simulink model "XROBO01_reference"  (R2025a)
settings: Solver=ode15s  StartTime=0  StopTime=2.95184041250516  MaxStep=0.002  RelTol=1e-3  AbsTol=1e-4  EnableMultiTasking=on
InitFcn:
  | d2r = pi/180; r2d = 180/pi;
  | assert(exist('initial_forward_speed_mps','var')==1,'XROBO01_PUBLIC_INPUT_MISSING:initial_forward_speed_mps');
  | assert(exist('supported_mass_kg','var')==1,'XROBO01_PUBLIC_INPUT_MISSING:supported_mass_kg');
  | assert(exist('ground_stiffness_npm','var')==1,'XROBO01_PUBLIC_INPUT_MISSING:ground_stiffness_npm');
  | assert(exist('ground_damping_nspm','var')==1,'XROBO01_PUBLIC_INPUT_MISSING:ground_damping_nspm');
  | assert(exist('propulsive_torque_nm','var')==1,'XROBO01_PUBLIC_INPUT_MISSING:propulsive_torque_nm');
  | assert(exist('knee_stiffness_nmprad','var')==1,'XROBO01_PUBLIC_INPUT_MISSING:knee_stiffness_nmprad');
  | u0 = initial_forward_speed_mps; M = supported_mass_kg;
  | ground = struct('stiffness',ground_stiffness_npm,'damping',ground_damping_nspm);
  | Trq_propulsive = propulsive_torque_nm; k2 = knee_stiffness_nmprad;
model workspace (MAT data in the model file):
  DataValues = [0 -8.46607862487e-28 -3.0230079043e-07 -3.0230079043e-07 -0.00122724595841 -0.00736196406339 -0.038035529735 -0.172846716535 -0.307649006025 -0.442435463868 -0.577199164336 -0.711933194065 ... (996 elements, 996x1)]
  F90_INTERNAL_TASK_VERSION = "F90-XROBO-01/INTERNAL_TESTABLE_V0"
  J = 0.317042404181
  L = 1
  L_back = 1.5
  L_stance = 0.85
  N = 80
  T_cg = 0.491973402084
  T_stance = 0.243620261167
  TimeValues = [0 6.27984023631e-30 2.24236125286e-09 2.24236125286e-09 9.10328015658e-06 5.46084691332e-05 0.000282134414016 0.00128213441402 0.00228213441402 0.00328213441402 0.00428213441402 0.00528213441402 ... (996 elements, 996x1)]
  bw = 200
  g = 9.81
  joint_damping = 0.1
  k = 5315
  knee_torque.time = [0 3.68781730895e-05 7.3756346179e-05 0.000110634519268 0.000347975944129 0.00058531736899 0.000822658793851 0.00106000021871 0.00146561022046 0.00187122022221 0.00227683022396 0.00268244022572 ... (1021 elements, 1021x1)]
  knee_torque.signals.values = [0.714762207266 1.14171505645 1.56256115584 1.97723731234 4.51139321024 6.81208984715 8.89224399956 10.7664604725 13.5316206084 15.8030887862 17.6429346124 19.1050336017 ... (1021 elements, 1021x1)]
  knee_torque.signals.dimensions = 1
  knee_torque.signals.label = ''
  knee_torque.signals.title = ''
  knee_torque.signals.plotStyle = 0
  knee_torque.blockName = 'sm_robot_run_03_leg_inverse_dyn/Knee Torque'
  l1 = 0.551688959481
  l2 = 0.551688959481
  leg_angle0 = -14.9486693308
  leg_vel0 = -106.091010331
  m = 25
  m1 = 1.1328847338
  m2 = 1.1328847338
  t_final = 2.95184041251
  t_th = [0 1.25e-05 2.5e-05 3.75e-05 8.75e-05 0.0001375 0.0001875 0.0002375 0.0004875 0.0007375 0.0009875 0.0012375 ... (751 elements, 751x1)]
  t_w = [0 1.25e-05 2.5e-05 3.75e-05 8.75e-05 0.0001375 0.0001875 0.0002375 0.0004875 0.0007375 0.0009875 0.0012375 ... (751 elements, 751x1)]
  th1 = 0.436332312999
  th1_0 = 0.691388219212
  th2 = 2.26892802759
  th2_0 = 1.75881621517
  th_dot0 = -108.218481968
  u_th = [11.0006741688 10.9993214378 10.9979687478 10.9966160991 10.9912058873 10.9857963249 10.9803874265 10.9749791998 10.9479483285 10.9209347423 10.8939387479 10.8669607548 ... (751 elements, 751x1)]
  u_w = [-108.221180812 -108.217887648 -108.214589671 -108.211286593 -108.198027643 -108.184691484 -108.171279404 -108.157793731 -108.089402099 -108.019570529 -107.948589122 -107.875696757 ... (751 elements, 751x1)]
  v0 = 0
  x0 = 0
  y0 = 0.85
values from neighbouring files (symbols this model uses):
  s = sin(q)    [Extr_Data_Cam_Roller_Curve.m]
undefined symbols (not defined in the file or in its folder): Extr_Data_Mesh, X, Y, Z
libraries: sm_lib x32, nesl_utility x10, fl_lib x5, sm_robot_run_4legs_lib x4, batteryecm_lib x1
(part 1 of 3)
CloseFcn:
  | try,close(h1_sm_robot_run_4legs),end
  | clear h1_sm_robot_run_4legs
  | try,close(h2_sm_robot_run_4legs),end
  | clear h2_sm_robot_run_4legs
  | try,close(h3_sm_robot_run_4legs),end
  | clear h3_sm_robot_run_4legs
  | try,close(h4_sm_robot_run_4legs),end
  | clear h4_sm_robot_run_4legs
  | 
  | 
  | clear simlog_sm_robot_run_4legs
  | clear logsout_sm_robot_run_4legs
Description:
  | Mechatronic Running Robot
  | 
  | Copyright 2012-2025 The MathWorks, Inc.
settings Model: Creator=rhyde  LastModifiedBy=SimuVerity Contributors
settings SolverCC: AutoScaleAbsTol=off  MaxConsecutiveZCs=10000  AlgebraicLoopSolver=TrustRegion
settings DataIOCC: MaxDataPoints=10000  SaveFinalState=on  SaveFormat=Array  SignalLoggingSaveFormat=ModelDataLogs  SaveState=on  SignalLoggingName=logsout_sm_robot_run_4legs  OutputTimes=[0:0.01:t_final]
settings OptimizationCC: ReuseModelBlockBuffer=off  ExpressionDepthLimit=2147483647.0  InitFltsAndDblsToZero=on  LifeSpan=inf
settings DebuggingCC: SaveWithParameterizedLinksMsg=none  UnderspecifiedInitializationDetection=Classic  MergeDetectMultiDrivingBlocksExec=none  SignalResolutionControl=TryResolveAllWithWarning  SolverPrmCheckMsg=warning  MultiTaskDSMMsg=warning  MultiTaskCondExecSysMsg=none  FcnCallInpInsideContextMsg=warning  UnconnectedInputMsg=warning  UnconnectedOutputMsg=warning  UnconnectedLineMsg=warning  StateNameClashWarn=warning  PregeneratedLibrarySubsystemCodeDiagnostic=none  SFUnexpectedBacktrackingDiag=warning  SFNoUnconditionalDefaultTransitionDiag=warning  SFExecutionAtInitializationDiag=none  ArithmeticOperatorsInVariantConditions=warning
settings HardwareCC: ProdBitPerPointer=32.0  ProdBitPerSizeT=32.0  ProdBitPerPtrDiffT=32.0  ProdLargestAtomicFloat=None  ProdIntDivRoundTo=Undefined  ProdEndianess=Unspecified  ProdWordSize=32.0  ProdHWDeviceType=32-bit Generic
settings ModelReferenceCC: EnableRefExpFcnMdlSchedulingChecks=on  PropagateSignalLabelsOutOfModel=off
settings SFSimCC: SimUseLocalCustomCode=off  SimParseCustomCode=off  CustomCodeUndefinedFunction=UseInterfaceOnly
settings RTWCC: RTWUseLocalCustomCode=off  GPUComputeCapability=3.5  DLArmComputeVersion=19.05
settings CodeAppCC: StateflowObjectComments=on
settings GRTTargetCC: TargetFcnLib=ansi_tfl_tmw.mat  TargetLangStandard=C89/C90 (ANSI)  CombineOutputUpdateFcns=off  GRTInterface=on
settings ConfigComp: CovMetricSettings=dw  CovSaveCumulativeToWorkspaceVar=on  CovSaveSingleToWorkspaceVar=on  CovExternalEMLEnable=off
settings SimscapeCC: SimscapeNormalizeSystem=off  SimscapeLogType=all  SimscapeLogSimulationStatistics=on  SimscapeLogName=simlog_sm_robot_run_4legs  SimscapeLogDataHistory=50000.0
settings ConfigurationSet: Description=SimMechanics 2G
settings DiagnosticsConfigSet: SimMechanicsUnconnectedFramePorts=none  SimMechanicsRigidlyBoundBlock=none
settings ExplorerConfigSet: InternalSimMechanicsExplorerSettings="<ExplorerConfiguration><canonicalview>default</canonicalview><AnimationSetting><BasePlaybackSpeed>1.0</BasePlaybackSpeed><PlaybackSpeedFactor>0.5</PlaybackSpeedFactor></AnimationSetting><TilePanel><TileInfo><Tiles Columns=\"1\" Count=\"1\" Rows=\"1\"><Column Weight=\"1\"/><Row Weight=\"1\"/><Tile Height=\"1\" Width=\"1\" X=\"0\" Y=\"0\"/></Tiles></TileInfo><SceneInfo><SceneViewer><BGColor><R>1</R><G>1</G><B>1</B></BGColor><Camera><DoPerspective>on</DoPerspective><Position><X>9.65055700274290018</X><Y>0.935000000000000053</Y><Z>1.00000000000000089</Z></Position><Center><X>8.79768847079045635</X><Y>0.76135182233306975</Y><Z>0.507596123493896711</Z></Center><Up><X>0</X><Y>1</Y><Z>0</Z></Up><ViewLimDist>1</ViewLimDist><YLim>0.466307658154998583</YLim><XLim>0.552660928183702049</XLim></Camera></SceneViewer></SceneInfo></TilePanel><MechEditorPanel><Cameras><Camera><Id>Camera1</Id><Value><Name>Body</Name><NativeCamera><PositionTrackingFeature>Body_Constraint.Camera.Transform_Camera.F</PositionTrackingFeature><CenterTrackingFeature>Body_Constraint.World_Frame.W</CenterTrackingFeature><UpVectorTrackingFeature>Body_Constraint.World_Frame.W</UpVectorTrackingFeature><CenterTrackingOrigin>off</CenterTrackingOrigin><CenterTrackingDirection>-Z</CenterTrackingDirection><UpVectorTrackingDirection>+Y</UpVectorTrackingDirection></NativeCamera></Value></Camera><Camera><Id>Camera2</Id><Value><Name>Body_Iso</Name><NativeCamera><PositionTrackingFeature>Body_Constraint.Camera.Transform_Camera_BodyIso.F</PositionTrackingFeature><CenterTrackingFeature>Body_Constraint.Camera.Transform_Camera_BodyIso_Aim.F</CenterTrackingFeature><UpVectorTrackingFeature>Body_Constraint.World_Frame.W</UpVectorTrackingFeature><CenterTrackingOrigin>off</CenterTrackingOrigin><CenterTrackingDirection>-Z</CenterTrackingDirection><UpVectorTrackingDirection>+Y</UpVectorTrackingDirection></NativeCamera></Value></Camera></Cameras><GfxPanelCameraMap><MapElement CameraMLId=\"Camera2\" GfxPanelIndex=\"0\"/></GfxPanelCameraMap><VideoCreator><PlaybackSpeedRatio>1.0</PlaybackSpeedRatio><FrameRate>30</FrameRate><VideoFormat>Motion JPEG AVI</VideoFormat><FrameSize>auto</FrameSize></VideoCreator></MechEditorPanel></ExplorerConfiguration>"

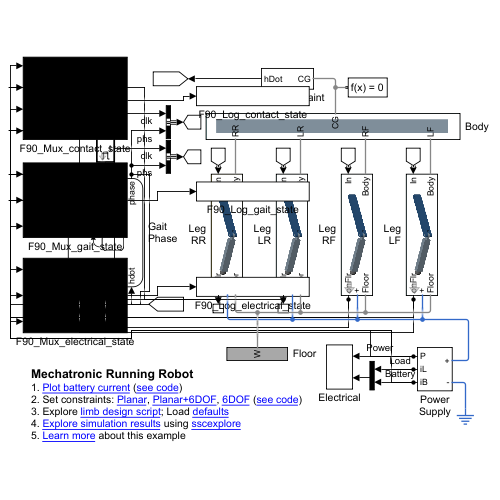
[thumbnail: Simulink's stored preview of the top-level diagram]
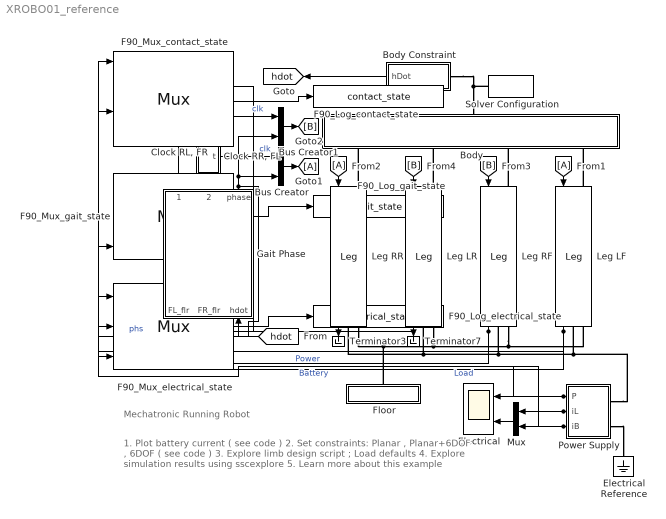
== system XROBO01_reference ==
  note: Mechatronic Running Robot
  note: 1. Plot battery current ( see code )
      | 2. Set constraints: Planar , Planar+6DOF , 6DOF ( see code )
      | 3. Explore limb design script ; Load defaults
      | 4. Explore simulation results using sscexplore
      | 5. Learn more about this example
  Body : Subsystem  Tag=CustomStyle
      mask Display: image('sm_robot_run_body_IMAGE.png')
  Body Constraint : Subsystem
  Bus Creator : BusCreator  Inputs=2
  Bus Creator1 : BusCreator  Inputs=2
  "Clock RL, FR" : Subsystem  TreatAsAtomicUnit=on  mask{t0=0}
      mask prompts: t0 "Initial local time"
  "Clock RR, FL" : Subsystem  TreatAsAtomicUnit=on  mask{t0=3*T_cg/4}
      mask prompts: t0 "Initial local time"
  Electrical : Scope  NumInputPorts=2
      settings: ActiveDisplayYMinimum=-181.58066  ActiveDisplayYMaximum=525.06229
  Electrical Reference : fl_lib/Electrical/Electrical Elements/Electrical Reference
  F90_Log_contact_state : ToWorkspace  VariableName=contact_state  SaveFormat=Timeseries  SampleTime=-1
  F90_Log_electrical_state : ToWorkspace  VariableName=electrical_state  SaveFormat=Timeseries  SampleTime=-1
  F90_Log_gait_state : ToWorkspace  VariableName=gait_state  SaveFormat=Timeseries  SampleTime=-1
  F90_Mux_contact_state : Mux
  F90_Mux_electrical_state : Mux  Inputs=3
  F90_Mux_gait_state : Mux  Inputs=3
  Floor : Subsystem
  From1 : From
  From2 : From
  Gait Phase : Stateflow chart  Tag=PublishSubsystem  TreatAsAtomicUnit=on
  Goto1 : Goto
  Leg LF : sm_robot_run_4legs_lib/Leg  Tag=PublishSubsystemCustomStyle  leg_type=Front Left  leg_width=0.1*l1  th1_0=d2r*u_th(find(t_th > 3*T_cg/4,1))  th2_0=-50*d2r+th2  th1_dot_0=-d2r*u_w(find(t_th > 3*T_cg/4,1))  x0=L_back  popup_contact_model=Planar
  Leg LR : sm_robot_run_4legs_lib/Leg  Tag=CustomStyle  leg_type=Rear Left  leg_width=0.1*l1  th1_0=th1_0  th2_0=th2_0  th1_dot_0=u0/L_stance  x0=0  popup_contact_model=Planar
  Leg RF : sm_robot_run_4legs_lib/Leg  Tag=CustomStyle  leg_type=Front Right  leg_width=0.1*l1  th1_0=th1_0  th2_0=th2_0  th1_dot_0=u0/L_stance  x0=L_back  popup_contact_model=Planar
  Leg RR : sm_robot_run_4legs_lib/Leg  Tag=CustomStyle  leg_type=Rear Right  leg_width=0.1*l1  th1_0=d2r*u_th(find(t_th > 3*T_cg/4,1))  th2_0=-50*d2r+th2  th1_dot_0=-d2r*u_w(find(t_th > 3*T_cg/4,1))  x0=0  popup_contact_model=Planar
  Mux : Mux  Inputs=2
  Power Supply : Subsystem  Tag=PublishSubsystem
  Solver Configuration : nesl_utility/Solver Configuration  PhysicalDomain=network_engine_domain  SubClassName=solver  LeftPortType=input  RightPortType=generic  Tones=[]  Harmonics=[]  SimulateNoise=off  Profile=off  UseLocalSampling=off  EnableSwitchedLinearOptims=on  FrequencyDomain=off  UseCCode=off  RelTol=0.001  AbsTol=1e-06  MinStep=1e-09  ToWorkspace=off  RevertToSquareIcSolve=off  NumHomotopyIterations=100  PhasorMode=off  PhasorModeNumHarmonics=1  ConsistencySolver=NEWTON_FTOL  IndexReductionMethod=DerivativeReplacement  DoDC=off  ResidualTolerance=1e-9  ConsistencyTolSource=GLOBAL  ConsistencyAbsTol=0.001  ConsistencyRelTol=0.001  ConsistencyTolFactor=0.001  UseLocalSolver=off  LocalSolverChoice=NE_BACKWARD_EULER_ADVANCER  ResolveIndetEquations=on  FunctionEvalNumThread=1  LocalSolverSampleTime=.001  DoFixedCost=off  MaxNonlinIter=12  MaxModeIter=2  ComputeImpulses=off  ImpulseIterations=2  LinearAlgebra=Sparse  LinearAlgebraNumThread=0  EquationFormulation=NE_TIME_EF  DelaysMemoryBudget=1024  AutomaticFiltering=on  FilteringTimeConstant=0.001  PartitionStorageMethod=AS_NEEDED  PartitionMemoryBudget=1024  PartitionMethod=FAST  MultibodyUseLocalSolver=off  MultibodyLocalSolverChoice=ODE1  MultibodyLocalSolverSampleTime=0.001
  Terminator3 : Terminator
  Terminator7 : Terminator
  tag scope: hdot=global
  wires:
  [hdot] -> Gait Phase/3(hdot)
  Leg RR/1 -> Terminator3/1, F90_Mux_contact_state/4
  Leg LF/1 -> Gait Phase/1(FL_flr), F90_Mux_contact_state/1
  Leg LR/1 -> Terminator7/1, F90_Mux_contact_state/2
  Gait Phase/1(RL_FR_aerial) -> "Clock RL, FR"/Enable, F90_Mux_gait_state/1
  Gait Phase/2(RR_FL_aerial) -> "Clock RR, FL"/Enable, F90_Mux_gait_state/2
  "Clock RR, FL"/1(t) -> Bus Creator/1  "clk"
  Leg RF/1 -> Gait Phase/2(FR_flr), F90_Mux_contact_state/3
  Power Supply/2(iL) -> Mux/1, F90_Mux_electrical_state/2  "Load"
  Power Supply/1(P) -> Electrical/1, F90_Mux_electrical_state/1  "Power"
  Bus Creator/1 -> Goto1/1
  Bus Creator1/1 -> [B]
  "Clock RL, FR"/1(t) -> Bus Creator1/1  "clk"
  Gait Phase/3(phase) -> Bus Creator1/2, Bus Creator/2, F90_Mux_gait_state/3  "phs"
  From1/1 -> Leg LF/1
  From2/1 -> Leg RR/1
  [B] -> Leg RF/1
  [B] -> Leg LR/1
  Body Constraint/1(hDot) -> [hdot]
  Mux/1 -> Electrical/2
  Power Supply/3(iB) -> Mux/2, F90_Mux_electrical_state/3  "Battery"
  F90_Mux_contact_state/1 -> F90_Log_contact_state/1
  F90_Mux_gait_state/1 -> F90_Log_gait_state/1
  F90_Mux_electrical_state/1 -> F90_Log_electrical_state/1
  connections:
  Body Constraint/LConn1 -- Solver Configuration/RConn1 -- Body/RConn1
  Power Supply/LConn2 -- Electrical Reference/LConn1
  Power Supply/LConn1 -- Leg RR/RConn1 -- Leg LR/RConn1 -- Leg RF/RConn1 -- Leg LF/RConn1
  Leg LF/LConn1 -- Body/LConn4
  Leg RF/LConn1 -- Body/LConn3
  Leg LR/LConn1 -- Body/LConn2
  Leg RR/LConn1 -- Body/LConn1
  Floor/RConn1 -- Leg LF/RConn2 -- Leg RF/RConn2 -- Leg LR/RConn2 -- Leg RR/RConn2
